simulink model "tb_dq_current_control"  (R2025b)
settings: Solver=VariableStepAuto  StartTime=0.0  StopTime=0.02  MaxStep=1e-5  RelTol=1e-6  AbsTol=1e-9
settings Model: Creator=semih  LastModifiedBy=semih

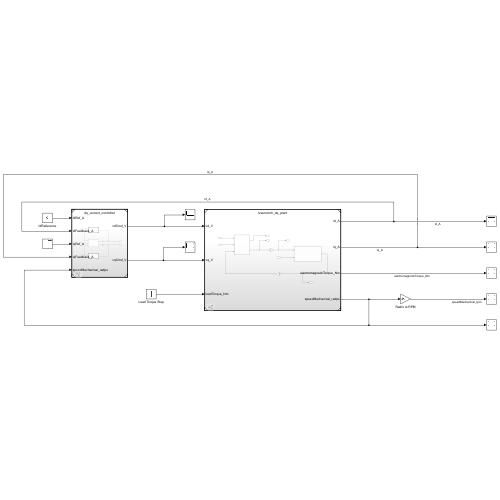
[thumbnail: Simulink's stored preview of the top-level diagram]
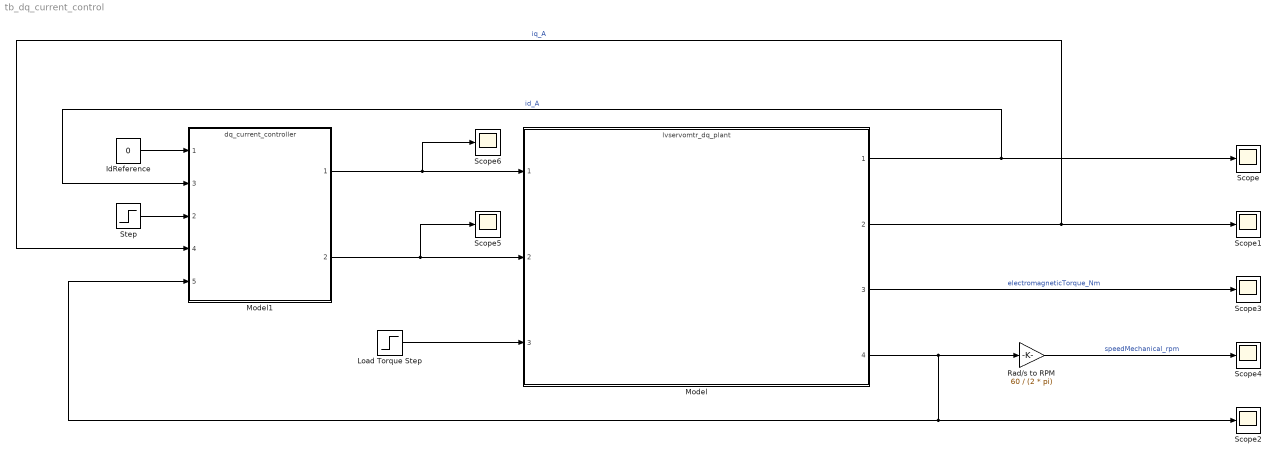
== system tb_dq_current_control ==
  IdReference : Constant  Value=0
  Load Torque Step : Step  Time=0.030  After=0  SampleTime=0
  Model : ModelReference  ModelNameDialog=lvservomtr_dq_plant  SimulationMode=Normal  ModelReferenceVersion=1.8
  Model1 : ModelReference  ModelNameDialog=dq_current_controller.slx  SimulationMode=Normal  ModelReferenceVersion=1.5
      settings: PortSchema="{\"entries\":[{\"content\":{\"sides\":[{\"content\":{\"connectorIds\":[\"In1\",\"In3\",\"In2\",\"In4\",\"In5\"]},\"type\":\"ConnectorPlacement.EquallySpacedRectSide\",\"uuid\":\"770debb9-2b2b-46a4-b6d4-b3cc8bc40512\"},{\"content\":{\"connectorIds\":[\"Out1\",\"Out2\"],\"side\":\"RIGHT\"},\"type\":\"ConnectorPlacement.EquallySpacedRectSide\",\"uuid\":\"10529b08-f942-4ed5-be6b-2ca61e24ccbd\"},{\"content\":{\"side\":\"TOP\"},\"type\":\"ConnectorPlacement.EquallySpacedRectSide\",\"uuid\":\"f8c183bf-1389-4593-9ed4-5d7ce061c30e\"}]},\"type\":\"ConnectorPlacement.EquallySpacedConnector\",\"uuid\":\"7720b2ba-7d08-46f0-a5d3-6c147234f35e\"}],\"packageUris\":[\"http://schema.mathworks.com/mf0/Connector/R2020b\"],\"version\":\"1.0\"}"
  Rad/s to RPM : Gain  Gain=60 / (2 * pi)
  Scope{,1..6} (7 alike) : Scope
      Scope settings: ActiveDisplayYMinimum=-0.032374393576631341  ActiveDisplayYMaximum=0.031833419479255054
      Scope1 settings: ActiveDisplayYMinimum=-0.63597233219420146  ActiveDisplayYMaximum=2.1211566623596005
      Scope2 settings: ActiveDisplayYMinimum=-14.648422716149396  ActiveDisplayYMaximum=131.83580444534459  DataLoggingVariableName=ScopeData2
      Scope3 settings: ActiveDisplayYMinimum=-0.060906186129986689  ActiveDisplayYMaximum=0.13304762379593027  DataLoggingVariableName=ScopeData3
      Scope4 settings: ActiveDisplayYMinimum=-3208.6952472436656  ActiveDisplayYMaximum=2366.4935888215819  DataLoggingVariableName=ScopeData4
      Scope5 settings: ActiveDisplayYMinimum=-0.57278929483551588  ActiveDisplayYMaximum=5.1551036535196442  DataLoggingVariableName=ScopeData5
      Scope6 settings: ActiveDisplayYMinimum=-0.29844789045009457  ActiveDisplayYMaximum=0.064252592645553649  DataLoggingVariableName=ScopeData6
  Step : Step  Time=0.005  After=2  SampleTime=0
  wires:
  Load Torque Step/1 -> Model/3
  Rad/s to RPM/1 -> Scope4/1  "speedMechanical_rpm"
  Model/4 -> Model1/5, Scope2/1, Rad/s to RPM/1
  Model1/2 -> Scope5/1, Model/2
  Model/3 -> Scope3/1  "electromagneticTorque_Nm"
  Model/1 -> Model1/3, Scope/1  "id_A"
  Model/2 -> Model1/4, Scope1/1  "iq_A"
  Step/1 -> Model1/2
  Model1/1 -> Scope6/1, Model/1
  IdReference/1 -> Model1/1
